simulink model "lcc3_comparison"  (R2024b)
settings: Solver=VariableStepAuto  StartTime=0.0  StopTime=0.016  RelTol=1e-3
InitFcn:
  | SIMSTEP=1e-8; Vin=50; Cs=135e-9; Ls=4.7e-6; Cp=27e-9; fs=280e3; Ron=1.0000000000000001e-05; Rd=1.0000000000000001e-05; Co=6.25e-6; td=0; Coss=0; n=4;
undefined symbols (not defined in the file): Vo_test
libraries: fl_lib x29, nesl_utility x21, ee_lib x15, spsOnDelayLib x6, spsMeanLib x2, spspowerguiLib x1
settings Model: Creator=amazing  LastModifiedBy=amazing

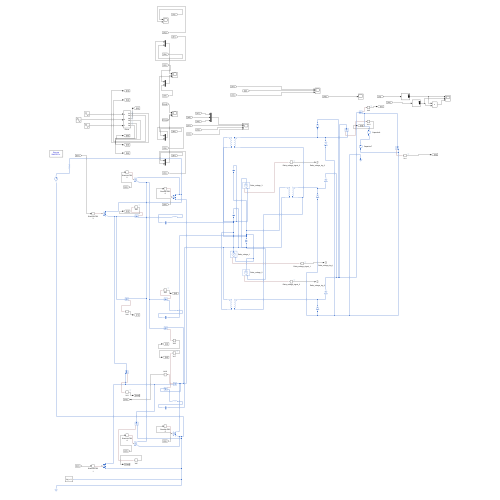
[thumbnail: Simulink's stored preview of the top-level diagram]
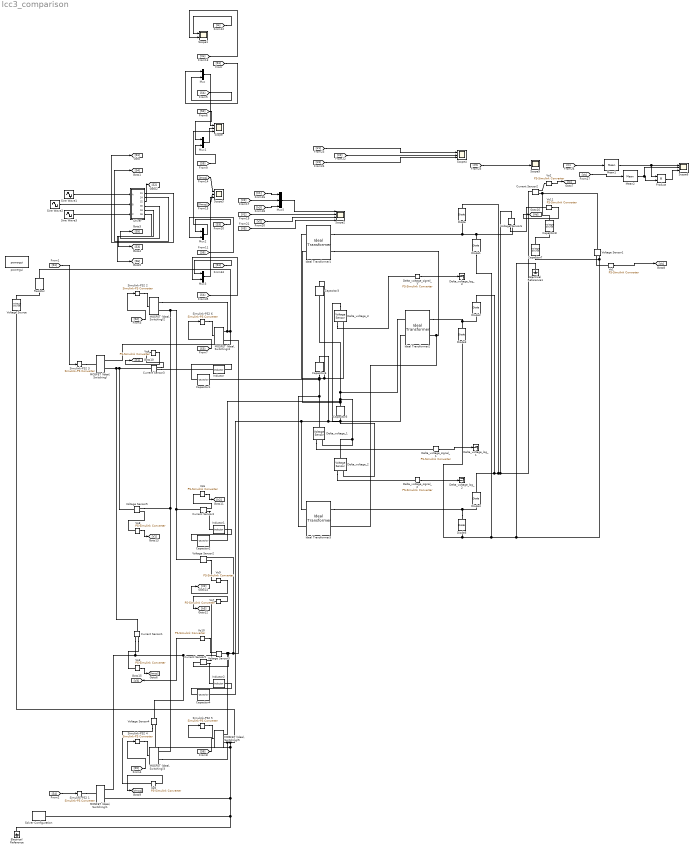
== system lcc3_comparison ==
  Capacitor1 : fl_lib/Electrical/Electrical Elements/Capacitor  c=Cs F  r=1.0000000000000001e-05 Ohm  g=0 1/Ohm  i_specify=off  i_priority=None  i=0 A  i_nominal_specify=off  i_nominal_value=1  i_nominal_unit=A  v_specify=off  v_priority=None  v=0 V  v_nominal_specify=off  v_nominal_value=1  v_nominal_unit=V  vc_specify=on  vc_priority=High  vc=0 V  vc_nominal_specify=off  vc_nominal_value=1  vc_nominal_unit=V
  Capacitor2 : fl_lib/Electrical/Electrical Elements/Capacitor  c=Cs F  r=1.0000000000000001e-05 Ohm  g=0 1/Ohm  i_specify=off  i_priority=None  i=0 A  i_nominal_specify=off  i_nominal_value=1  i_nominal_unit=A  v_specify=off  v_priority=None  v=0 V  v_nominal_specify=off  v_nominal_value=1  v_nominal_unit=V  vc_specify=on  vc_priority=High  vc=0 V  vc_nominal_specify=off  vc_nominal_value=1  vc_nominal_unit=V
  Capacitor3 : fl_lib/Electrical/Electrical Elements/Capacitor  c=Cp F  r=1.0000000000000001e-05 Ohm  g=0 1/Ohm  i_specify=off  i_priority=None  i=0 A  i_nominal_specify=off  i_nominal_value=1  i_nominal_unit=A  v_specify=off  v_priority=None  v=0 V  v_nominal_specify=off  v_nominal_value=1  v_nominal_unit=V  vc_specify=on  vc_priority=High  vc=0 V  vc_nominal_specify=off  vc_nominal_value=1  vc_nominal_unit=V
  Capacitor4 : fl_lib/Electrical/Electrical Elements/Capacitor  c=Cs F  r=1.0000000000000001e-05 Ohm  g=0 1/Ohm  i_specify=off  i_priority=None  i=0 A  i_nominal_specify=off  i_nominal_value=1  i_nominal_unit=A  v_specify=off  v_priority=None  v=0 V  v_nominal_specify=off  v_nominal_value=1  v_nominal_unit=V  vc_specify=on  vc_priority=High  vc=0 V  vc_nominal_specify=off  vc_nominal_value=1  vc_nominal_unit=V
  Capacitor5 : fl_lib/Electrical/Electrical Elements/Capacitor  c=Cp F  r=1.0000000000000001e-05 Ohm  g=0 1/Ohm  i_specify=off  i_priority=None  i=0 A  i_nominal_specify=off  i_nominal_value=1  i_nominal_unit=A  v_specify=off  v_priority=None  v=0 V  v_nominal_specify=off  v_nominal_value=1  v_nominal_unit=V  vc_specify=on  vc_priority=High  vc=0 V  vc_nominal_specify=off  vc_nominal_value=1  vc_nominal_unit=V
  Capacitor6 : fl_lib/Electrical/Electrical Elements/Capacitor  c=Cp F  r=1.0000000000000001e-05 Ohm  g=0 1/Ohm  i_specify=off  i_priority=None  i=0 A  i_nominal_specify=off  i_nominal_value=1  i_nominal_unit=A  v_specify=off  v_priority=None  v=0 V  v_nominal_specify=off  v_nominal_value=1  v_nominal_unit=V  vc_specify=on  vc_priority=High  vc=0 V  vc_nominal_specify=off  vc_nominal_value=1  vc_nominal_unit=V
  Capacitor7 : ee_lib/Sources/Voltage Source  dc_voltage=Vo_test/2 V  ac_voltage=0 V  ac_shift=0 rad  ac_frequency=60 Hz  noise_mode=ee.enum.sources.noise.Disabled  PSD=0 V^2/Hz  sample_time=1e-3 s  repeatability=ee.enum.sources.repeatability.NotRepeatable  user_seed=0  auto_seed=3890346746  i_specify=off  i_priority=None  i=0 A  i_nominal_specify=off  i_nominal_value=1  i_nominal_unit=A  v_specify=off  v_priority=None  v=0 V  v_nominal_specify=off  v_nominal_value=1  v_nominal_unit=V
  Capacitor8 : ee_lib/Sources/Voltage Source  dc_voltage=Vo_test/2 V  ac_voltage=0 V  ac_shift=0 rad  ac_frequency=60 Hz  noise_mode=ee.enum.sources.noise.Disabled  PSD=0 V^2/Hz  sample_time=1e-3 s  repeatability=ee.enum.sources.repeatability.NotRepeatable  user_seed=0  auto_seed=3499211588  i_specify=off  i_priority=None  i=0 A  i_nominal_specify=off  i_nominal_value=1  i_nominal_unit=A  v_specify=off  v_priority=None  v=0 V  v_nominal_specify=off  v_nominal_value=1  v_nominal_unit=V
  Current Sensor{1..5} (5 alike) : fl_lib/Electrical/Electrical Sensors/Current Sensor
  Delta_voltage_1 : fl_lib/Electrical/Electrical Sensors/Voltage Sensor
  Delta_voltage_2 : fl_lib/Electrical/Electrical Sensors/Voltage Sensor
  Delta_voltage_3 : fl_lib/Electrical/Electrical Sensors/Voltage Sensor
  Delta_voltage_log_1 : Terminator
  Delta_voltage_log_2 : Terminator
  Delta_voltage_log_3 : Terminator
  Delta_voltage_signal_1 : nesl_utility/PS-Simulink Converter  PhysicalDomain=network_engine_domain  SubClassName=ps_output  LeftPortType=input  RightPortType=output  PseudoPeriodic=off  Frequencies=[]  VectorFormat=inherit  Unit=inherit  AffineConversion=off
  Delta_voltage_signal_2 : nesl_utility/PS-Simulink Converter  PhysicalDomain=network_engine_domain  SubClassName=ps_output  LeftPortType=input  RightPortType=output  PseudoPeriodic=off  Frequencies=[]  VectorFormat=inherit  Unit=inherit  AffineConversion=off
  Delta_voltage_signal_3 : nesl_utility/PS-Simulink Converter  PhysicalDomain=network_engine_domain  SubClassName=ps_output  LeftPortType=input  RightPortType=output  PseudoPeriodic=off  Frequencies=[]  VectorFormat=inherit  Unit=inherit  AffineConversion=off
  Diode{,1..5} (6 alike) : ee_lib/Semiconductors & Converters/Diode  ModelType=ee.enum.diode.modelType.pwl  TableType=ee.enum.diode.tableType.IfMat  IfMat=[.07, .12, .19, 1.75, 4.24, 7.32, 11.2; .16, .3, .72, 2.14, 5.02, 8.35, 13.12] A  VfMat=[.9, 1.15, 1.25, 1.5, 1.75, 2.17, 2.6, 2.85; .58, .68, .75, 1.1, 1.38, 1.77, 2.27, 2.7] V  TjVec=[25, 125] degC  VfVec=[.5, .7, .9, 1.3, 1.7, 2.1, 2.5] V  IfVec=[.1, .2, .5, 1, 2, 4, 7, 10] A  IrMat=[1e-06, 2e-06, 5e-06, 1e-05, 2.5e-05, 5e-05, .0001; 2e-06, 5e-06, 1e-05, 4e-05, 8e-05, .0002, .0005] A  VrMat=[10, 100, 200, 250, 300, 325, 350; 10, 70, 160, 220, 270, 300, 320] V  VrVec=[10, 20, 40, 50, 70, 80, 100] V  IrVec=[1e-06, 2e-06, 5e-06, 1e-05, 2e-05, 5e-05, .0001] A  Vf=9.9999999999999995e-07 V  Ron=1.0000000000000001e-05 Ohm  Goff=1e-10 S  prmExp=ee.enum.diode.expParam.useTwo  I12=[.0137, .545] A  V12=[.6, .7] V  RS=0 Ohm  Tmeas=298.15 K  IS=1e-12 A  ec=1  I1=0.0137 A  V1=0.6 V  N_series=1  N_parallel=1  ZenerEnable=false  Rz=0.3 Ohm  BV=inf V  C_param=ee.enum.diode.capParam.fixed  CJ=0 pF  CJ0=5 pF  Vvec=[.1, 10, 100] V  Cvec=[3.5, 1, .4] pF  VJ=1 V  Mgrad=0.5  FC=0.5  Q_param=ee.enum.diode.recoveryParam.off  iRM=-7.15 A  iF=4 A  didt=-750 A/us  trr_factor=3  trr=115 ns  Qrr=150 nA*s  Vr=-600 V  Ls=150 nH  Erec=0.03 J  TT=50 ns  tau=100 ns  T_param=ee.enum.diode.temperatureParam.off  Tdevice=298.15 K  I1_T2=0.245 A  V1_T2=0.5 V  IS_T2=1.25e-7 A  Tmeas2=125 degC  XTI_param=ee.enum.diode.xtiParam.pn  XTI=3  EG_param=ee.enum.diode.egapParam.material_si  EG=1.11 eV  dBVdT=0 V/K  fault_action=simscape.enum.assert.action.none  t_fault=inf s  enable_fault_input=simscape.enum.onoff.off  i_specify=off  i_priority=None  i=0 A  i_nominal_specify=off  i_nominal_value=1  i_nominal_unit=A  v_specify=off  v_priority=None  v=0 V  v_nominal_specify=off  v_nominal_value=1  v_nominal_unit=V  v_capacitor_specify=off  v_capacitor_priority=None  v_capacitor=0 V  v_capacitor_nominal_specify=off  v_capacitor_nominal_value=1  v_capacitor_nominal_unit=V  Qj_specify=off  Qj_priority=High  Qj=0 C  Qj_nominal_specify=off  Qj_nominal_value=1  Qj_nominal_unit=C  i_diode_specify=off  i_diode_priority=None  i_diode=0 A  i_diode_nominal_specify=off  i_diode_nominal_value=1  i_diode_nominal_unit=A  v_diode_specify=off  v_diode_priority=None  v_diode=0 V  v_diode_nominal_specify=off  v_diode_nominal_value=1  v_diode_nominal_unit=V  i_capacitor_specify=off  i_capacitor_priority=None  i_capacitor=0 A  i_capacitor_nominal_specify=off  i_capacitor_nominal_value=1  i_capacitor_nominal_unit=A  power_dissipated_specify=off  power_dissipated_priority=None  power_dissipated=0 W  power_dissipated_nominal_specify=off  power_dissipated_nominal_value=1  power_dissipated_nominal_unit=W  fidelity_level=ee.enum.diode.fidelity.includeChargeDyn  rec_loss_model=ee.enum.diode.reverseRecoveryModel.fixed  ErecVal=0 J  scaleWithIandV=true  ErecMat=zeros(2, 3) J  TjrecVec=[298.15, 398.15] K  IfrecVec=[.1, 1, 10] A  IrecVal=10 A  VrecVal=10 V  tFilter=1 / 1000 / 100 s  thermal_network_parameterization=ee.enum.thermalNetworkTopology.junctionCase  Rth=[0, 10] K/W  Rth_Cauer=[1, 3, 10] K/W  Rth_Foster=[.08, .14, .22, .16] K/W  thermal_mass_parameterization=ee.enum.thermalNetwork.timeconstant  thermal_mass=[0, 1] J/K  thermal_mass_Cauer=[.1, .3, 1] J/K  thermal_mass_Foster=[.001, .005, .05, .5] J/K  thermal_time_constant=[0, 10] s  thermal_time_constant_Cauer=[1, 3, 10] s  thermal_time_constant_Foster=[7e-05, .0007, .01, .08] s  thermal_mass_initial_temperatures=[25, 25] degC  thermal_mass_initial_temperatures_Cauer=[25, 25, 25] degC  junction_thermal_mass=0.01 J/K  Tvec_initial_Foster=[25, 25, 25, 25] degC  no_thermal_network=0  junction_temperature_specify=off  junction_temperature_priority=None  junction_temperature=25 degC  junction_temperature_nominal_specify=off  junction_temperature_nominal_value=1  junction_temperature_nominal_unit=degC
  Driver : Subsystem
  Electrical Reference : fl_lib/Electrical/Electrical Elements/Electrical Reference
  Electrical Reference1 : fl_lib/Electrical/Electrical Elements/Electrical Reference
  Ideal Transformer1 : fl_lib/Electrical/Electrical Elements/Ideal Transformer  n=1/n  i1_specify=off  i1_priority=None  i1=0 A  i1_nominal_specify=off  i1_nominal_value=1  i1_nominal_unit=A  v1_specify=off  v1_priority=None  v1=0 V  v1_nominal_specify=off  v1_nominal_value=1  v1_nominal_unit=V  i2_specify=off  i2_priority=None  i2=0 A  i2_nominal_specify=off  i2_nominal_value=1  i2_nominal_unit=A  v2_specify=off  v2_priority=None  v2=0 V  v2_nominal_specify=off  v2_nominal_value=1  v2_nominal_unit=V
  Ideal Transformer2 : fl_lib/Electrical/Electrical Elements/Ideal Transformer  n=1/n  i1_specify=off  i1_priority=None  i1=0 A  i1_nominal_specify=off  i1_nominal_value=1  i1_nominal_unit=A  v1_specify=off  v1_priority=None  v1=0 V  v1_nominal_specify=off  v1_nominal_value=1  v1_nominal_unit=V  i2_specify=off  i2_priority=None  i2=0 A  i2_nominal_specify=off  i2_nominal_value=1  i2_nominal_unit=A  v2_specify=off  v2_priority=None  v2=0 V  v2_nominal_specify=off  v2_nominal_value=1  v2_nominal_unit=V
  Ideal Transformer3 : fl_lib/Electrical/Electrical Elements/Ideal Transformer  n=1/n  i1_specify=off  i1_priority=None  i1=0 A  i1_nominal_specify=off  i1_nominal_value=1  i1_nominal_unit=A  v1_specify=off  v1_priority=None  v1=0 V  v1_nominal_specify=off  v1_nominal_value=1  v1_nominal_unit=V  i2_specify=off  i2_priority=None  i2=0 A  i2_nominal_specify=off  i2_nominal_value=1  i2_nominal_unit=A  v2_specify=off  v2_priority=None  v2=0 V  v2_nominal_specify=off  v2_nominal_value=1  v2_nominal_unit=V
  Inductor : fl_lib/Electrical/Electrical Elements/Inductor  l=Ls H  r=1.0000000000000001e-05 Ohm  g=1e-10 1/Ohm  i_specify=off  i_priority=None  i=0 A  i_nominal_specify=off  i_nominal_value=1  i_nominal_unit=A  v_specify=off  v_priority=None  v=0 V  v_nominal_specify=off  v_nominal_value=1  v_nominal_unit=V  i_L_specify=on  i_L_priority=High  i_L=0 A  i_L_nominal_specify=off  i_L_nominal_value=1  i_L_nominal_unit=A
  Inductor1 : fl_lib/Electrical/Electrical Elements/Inductor  l=Ls H  r=1.0000000000000001e-05 Ohm  g=1e-10 1/Ohm  i_specify=off  i_priority=None  i=0 A  i_nominal_specify=off  i_nominal_value=1  i_nominal_unit=A  v_specify=off  v_priority=None  v=0 V  v_nominal_specify=off  v_nominal_value=1  v_nominal_unit=V  i_L_specify=on  i_L_priority=High  i_L=0 A  i_L_nominal_specify=off  i_L_nominal_value=1  i_L_nominal_unit=A
  Inductor2 : fl_lib/Electrical/Electrical Elements/Inductor  l=Ls H  r=1.0000000000000001e-05 Ohm  g=1e-10 1/Ohm  i_specify=off  i_priority=None  i=0 A  i_nominal_specify=off  i_nominal_value=1  i_nominal_unit=A  v_specify=off  v_priority=None  v=0 V  v_nominal_specify=off  v_nominal_value=1  v_nominal_unit=V  i_L_specify=on  i_L_priority=High  i_L=0 A  i_L_nominal_specify=off  i_L_nominal_value=1  i_L_nominal_unit=A
  MOSFET (Ideal, Switching){,1..5} (6 alike) : ee_lib/Semiconductors & Converters/MOSFET (Ideal, Switching)  port_option=ee.enum.controlport.ps  Rds=1.0000000000000001e-05 Ohm  Goff=1e-10 1/Ohm  Vth=2 V  diode_param=ee.enum.semiconductors.protectionDiode.external  diode_Vf=1e-9 V  diode_Ron=1e-9 Ohm  diode_Goff=1e-12 1/Ohm  diode_C=50e-9 F  diode_iRM=-235 A  diode_iF=300 A  diode_idot=-50 A/us  diode_trr_param=ee.enum.converters.diodeReverseParam.trr_factor  diode_trr_factor=3  diode_trr=15 us  diode_Qrr=1500 s*uA  ids_specify=off  ids_priority=None  ids=0 A  ids_nominal_specify=off  ids_nominal_value=1  ids_nominal_unit=A  vds_specify=off  vds_priority=None  vds=0 V  vds_nominal_specify=off  vds_nominal_value=1  vds_nominal_unit=V  vgs_specify=off  vgs_priority=None  vgs=0 V  vgs_nominal_specify=off  vgs_nominal_value=1  vgs_nominal_unit=V  thermal_loss_option=ee.enum.converters.thermalLossOption.constantvalues  Von_data=[0, 1.8, 3.2, 6, 10, 16; 0, 2, 5.5, 9.5, 15, 25] V  Tj=[298.15, 448.15] K  Iout_data=[0, 20, 40, 60, 80, 100] A  Eon_data=[0, 55.04, 124.57, 235.53, 362.12; 0, 71.25, 161.25, 304.88, 468.75] * 1e-6 J  Eoff_data=[0, 18, 30, 56.1, 76.5; 0, 22.5, 37.5, 70.13, 95.63] * 1e-6 J  Eon_data_3D=[zeros(2, 5, 3)] J  Eoff_data_3D=[zeros(2, 5, 3)] J  Tj_loss=[298.15, 448.15] K  Iout_data_loss=[0, 10, 20, 30, 40] A  tabulateWithVds=false  Vds_loss=[0, 150, 300] V  Eon_scalar=22.86e-3 J  Eoff_scalar=17.14e-3 J  Voff=300 V  Iout_scalar=600 A  useCurrentFromPreviousCycle=false  useVoltageFromPreviousCycle=false  diodeModelType=ee.enum.converters.diodeModelType.pwl  diodeTableType=ee.enum.diode.tableType.IfMat  diode_ReverseIVType=ee.enum.diode.diodeReverseIV.constant  diode_IfMat=[.07, .12, .19, 1.75, 4.24, 7.32, 11.2; .16, .3, .72, 2.14, 4.02, 6.35, 9.12] A  diode_VfMat=[.9, 1.15, 1.25, 1.5, 1.75, 2.17, 2.6, 2.85; .58, .68, .75, 1.1, 1.38, 1.77, 2.27, 2.7] V  diode_TjVec=[25, 125] degC  diode_VfVec=[.5, .7, .9, 1.3, 1.7, 2.1, 2.5] V  diode_IfVec=[.1, .2, .5, 1, 2, 4, 7, 10] A  diode_IrMat=[1e-06, 2e-06, 5e-06, 1e-05, 2.5e-05, 5e-05, .0001; 2e-06, 5e-06, 1e-05, 4e-05, 8e-05, .0002, .0005] A  diode_VrMat=[10, 100, 200, 250, 300, 325, 350; 10, 70, 160, 220, 270, 300, 320] V  diode_VrVec=[10, 20, 40, 50, 70, 80, 100] V  diode_IrVec=[1e-06, 2e-06, 5e-06, 1e-05, 2e-05, 5e-05, .0001] A  diode_Vr=-600 V  diode_Ls=150 nH  diode_Erec=0.03 J  diode_rec_loss_model=ee.enum.diode.reverseRecoveryModel.fixed  diode_ErecVal=0 J  diode_scaleWithIandV=true  diode_ErecMat=zeros(2, 3) J  diode_TjrecVec=[298.15, 398.15] K  diode_IfrecVec=[.1, 1, 10] A  diode_IrecVal=10 A  diode_VrecVal=10 V  diode_tFilter=1 / 1000 / 100 s  separateThermalPortForDiode=false  thermal_network_parameterization=ee.enum.thermalNetworkTopology.external  Rth=[.03, .2] K/W  Rth_Cauer=[.03, .1, .2] K/W  Rth_Foster=[.08, .14, .22, .16] K/W  thermal_mass_parameterization=ee.enum.thermalNetwork.timeconstant  thermal_mass=[3, 25] J/K  thermal_mass_Cauer=[3, 10, 25] J/K  thermal_mass_Foster=[.001, .005, .05, .5] J/K  thermal_time_constant=[.1, 5] s  thermal_time_constant_Cauer=[.1, 1, 5] s  thermal_time_constant_Foster=[7e-05, .0007, .01, .08] s  thermal_mass_initial_temperatures=[25, 25] degC  thermal_mass_initial_temperatures_Cauer=[25, 25, 25] degC  junction_thermal_mass=0.1 J/K  Tvec_initial_Foster=[25, 25, 25, 25] degC  RthDiode=[.03, .2] K/W  RthCauerDiode=[.03, .1, .2] K/W  RthFosterDiode=[.03, .2] K/W  thermalMassDiode=[3, 25] J/K  thermalMassCauerDiode=[3, 10, 25] J/K  thermalMassFosterDiode=[33, 50] J/K  thermalTauDiode=[.1, 5] s  thermalTauCauerDiode=[.1, 1, 5] s  thermalTauFosterDiode=[1, 10] s  thermalMassInitTempDiode=[25, 25] degC  thermalMassInitTempCauerDiode=[25, 25, 25] degC  junctionthermalMassDiode=0.1 J/K  TVecInitialFosterDiode=[25, 25, 25, 25] degC  no_thermal_network=0  mosfet_junction_temperature_specify=off  mosfet_junction_temperature_priority=None  mosfet_junction_temperature=25 degC  mosfet_junction_temperature_nominal_specify=off  mosfet_junction_temperature_nominal_value=1  mosfet_junction_temperature_nominal_unit=degC  diode_junction_temperature_specify=off  diode_junction_temperature_priority=None  diode_junction_temperature=25 degC  diode_junction_temperature_nominal_specify=off  diode_junction_temperature_nominal_value=1  diode_junction_temperature_nominal_unit=degC  Qj_specify=off  Qj_priority=None  Qj=0 W  Qj_nominal_specify=off  Qj_nominal_value=1  Qj_nominal_unit=W  accumulatedSwitchingLosses_specify=off  accumulatedSwitchingLosses_priority=None  accumulatedSwitchingLosses=0 J
  Mean1 : spsMeanLib/Mean  Freq=100e3  Vinit=0  Ts=0
  Mean2 : spsMeanLib/Mean  Freq=100e3  Vinit=0  Ts=0
  Mux{,1..3} (4 alike) : Mux  Inputs=2
  Mux5 : Mux  Inputs=3
  Product : Product
  Resistor : fl_lib/Electrical/Electrical Elements/Resistor  R=1.0000000000000001e-05 Ohm  i_specify=off  i_priority=None  i=0 A  i_nominal_specify=off  i_nominal_value=1  i_nominal_unit=A  v_specify=off  v_priority=None  v=0 V  v_nominal_specify=off  v_nominal_value=1  v_nominal_unit=V
  Scope{,3..4,6} (4 alike) : Scope  NumInputPorts=3
  Scope1 : Scope  NumInputPorts=2
  Scope2 : Scope  NumInputPorts=4
  Scope5 : Scope
  Simulink-PS2 {1..6} (6 alike) : nesl_utility/Simulink-PS Converter  PhysicalDomain=network_engine_domain  SubClassName=ps_input  LeftPortType=input  RightPortType=output  PseudoPeriodic=off  Frequencies=[]  NoiseDistribution=none  NoiseParameters=[]  Unit=1  AffineConversion=off  FilteringAndDerivatives=provide  SimscapeFilterOrder=1  InputFilterTimeConstant=0.001  UdotUserProvided=0
  Sine Wave1 : Sin  Frequency=2*pi*fs  SampleTime=0
  Sine Wave2 : Sin  Frequency=2*pi*fs  Phase=2*pi/3  SampleTime=0
  Sine Wave3 : Sin  Frequency=2*pi*fs  Phase=4*pi/3  SampleTime=0
  Solver Configuration : nesl_utility/Solver Configuration  PhysicalDomain=network_engine_domain  SubClassName=solver  LeftPortType=input  RightPortType=generic  Tones=[]  Harmonics=[]  SimulateNoise=off  Profile=off  UseLocalSampling=off  EnableSwitchedLinearOptims=on  FrequencyDomain=off  UseCCode=off  RelTol=0.001  AbsTol=0.001  MinStep=1e-09  ToWorkspace=off  RevertToSquareIcSolve=off  NumHomotopyIterations=100  PhasorMode=off  PhasorModeNumHarmonics=1  ConsistencySolver=NEWTON_XTOL_AFTER_FTOL  IndexReductionMethod=DerivativeReplacement  DoDC=off  ResidualTolerance=1e-09  ConsistencyTolSource=GLOBAL  ConsistencyAbsTol=0.001  ConsistencyRelTol=0.001  ConsistencyTolFactor=0.001  UseLocalSolver=off  LocalSolverChoice=NE_BACKWARD_EULER_ADVANCER  ResolveIndetEquations=on  FunctionEvalNumThread=1  LocalSolverSampleTime=0.001  DoFixedCost=off  MaxNonlinIter=3  MaxModeIter=2  ComputeImpulses=off  ImpulseIterations=2  LinearAlgebra=auto  LinearAlgebraNumThread=0  EquationFormulation=NE_TIME_EF  DelaysMemoryBudget=1024  AutomaticFiltering=on  FilteringTimeConstant=0.001  PartitionStorageMethod=AS_NEEDED  PartitionMemoryBudget=1024  PartitionMethod=ROBUST  MultibodyUseLocalSolver=off  MultibodyLocalSolverChoice=ODE1  MultibodyLocalSolverSampleTime=0.001
  Vo{1..11} (11 alike) : nesl_utility/PS-Simulink Converter  PhysicalDomain=network_engine_domain  SubClassName=ps_output  LeftPortType=input  RightPortType=output  PseudoPeriodic=off  Frequencies=[]  VectorFormat=inherit  Unit=inherit  AffineConversion=off
  Voltage Sensor{1..6} (6 alike) : fl_lib/Electrical/Electrical Sensors/Voltage Sensor
  Voltage Source : ee_lib/Sources/Voltage Source  dc_voltage=Vin V  ac_voltage=0 V  ac_shift=0 rad  ac_frequency=0 Hz  noise_mode=ee.enum.sources.noise.Disabled  PSD=0 V^2/Hz  sample_time=1e-3 s  repeatability=ee.enum.sources.repeatability.NotRepeatable  user_seed=0  auto_seed=3890346746  i_specify=off  i_priority=None  i=0 A  i_nominal_specify=off  i_nominal_value=1  i_nominal_unit=A  v_specify=off  v_priority=None  v=0 V  v_nominal_specify=off  v_nominal_value=1  v_nominal_unit=V
  powergui : spspowerguiLib/powergui  Priority=1  SimulationMode=Discrete  SampleTime=SIMSTEP  frequency=60  Iterations=50  frequencyindice=60  Pbase=100e6  ErrMax=1e-4  UnitsV=kV  UnitsW=MW  buscounter=0  FunctionMessages=off  echomessages=off  EnableUseOfTLC=off  CurrentSourceSwitches=off  DisableSnubberDevices=off  DisableRonSwitches=off  DisableVfSwitches=off  DisplayEquations=off  AutomaticDiscreteSolvers=off  SolverType=Tustin/Backward Euler (TBE)  Interpol=off  ExternalGateDelay=off  methode=off  Ts=100  x0status=blocks  SPID=on  SwTol=0  HookPort=off  NonlinearTolerance=1e-4  nMaxIteration=100  ContinueOnMaxIteration=off  RestoreLinks=warning  ResistiveCurrentMeasurement=off  Frange=[0:2:500]  Ylog=off  Xlog=on  ShowGrid=off  save=off  variable=ZData  structure=0  ZoomFFT=off  StartTime=0.0  cycles=1  DisplayStyle=1  fundamental=60  FreqAxis=off  MaxFrequency=1000  frequencyindicesteady=1  RmsSteady=1  display=off
  wires:
  Delta_voltage_signal_3/1 -> Delta_voltage_log_3/1
  Delta_voltage_signal_2/1 -> Delta_voltage_log_2/1
  Delta_voltage_signal_1/1 -> Delta_voltage_log_1/1
  [S1] -> Mux3/1
  [S4] -> Mux3/2
  Mux3/1 -> Scope3/3
  [Vd] -> Scope5/1
  Vo11/1 -> [Vd]
  Product/1 -> Scope6/3
  Mean2/1 -> Scope6/2, Product/2
  [Vo] -> Mean2/1
  Mean1/1 -> Product/1, Scope6/1
  [Io] -> Mean1/1
  [Ir3] -> Scope4/3
  [Ir1] -> Scope4/1
  [Ir2] -> Scope4/2
  [Vmos] -> Scope3/2
  [Imos] -> Scope3/1
  Vo5/1 -> [Vmos]
  [S5] -> Simulink-PS2 4/1
  Vo3/1 -> [Imos]
  [Vo] -> Scope1/2
  [Io] -> Scope1/1
  Mux5/1 -> Scope2/1
  [V2] -> Scope2/3
  [V3] -> Scope2/4
  [V1] -> Scope2/2
  Vo10/1 -> [V3]
  Vo9/1 -> [V2]
  Vo8/1 -> [V1]
  [Ir3] -> Mux5/3
  [Ir2] -> Mux5/2
  [Ir1] -> Mux5/1
  Vo7/1 -> [Ir3]
  Vo6/1 -> [Ir2]
  Vo4/1 -> [Ir1]
  Mux2/1 -> Scope/3
  Mux/1 -> Scope/1
  Mux1/1 -> Scope/2
  [S6] -> Mux2/2
  [S3] -> Mux2/1
  [S2] -> Mux1/1
  [S5] -> Mux1/2
  [S4] -> Mux/2
  [S1] -> Mux/1
  Vo2/1 -> [Io]
  Vo1/1 -> [Vo]
  [S3] -> Simulink-PS2 6/1
  [S6] -> Simulink-PS2 5/1
  [S2] -> Simulink-PS2 2/1
  [S4] -> Simulink-PS2 1/1
  [S1] -> Simulink-PS2 3/1
  Driver/6(S6) -> [S6]
  Driver/5(S3) -> [S3]
  Driver/4(S5) -> [S5]
  Driver/3(S2) -> [S2]
  Sine Wave3/1 -> Driver/3(C)
  Sine Wave2/1 -> Driver/2(B)
  Driver/2(S4) -> [S4]
  Sine Wave1/1 -> Driver/1(A)
  Driver/1(S1) -> [S1]
  connections:
  Delta_voltage_3/RConn1 -- Delta_voltage_signal_3/LConn1
  Delta_voltage_2/RConn1 -- Delta_voltage_signal_2/LConn1
  Delta_voltage_1/RConn1 -- Delta_voltage_signal_1/LConn1
  Capacitor7/LConn1 -- Capacitor8/RConn1
  Current Sensor2/RConn2 -- Voltage Sensor1/LConn1 -- Capacitor8/LConn1
  Voltage Sensor6/RConn1 -- Vo11/LConn1
  Vo6/LConn1 -- Current Sensor4/RConn1
  Voltage Sensor4/RConn1 -- Vo5/LConn1
  Current Sensor1/RConn1 -- Vo3/LConn1
  "MOSFET (Ideal, Switching)1"/RConn1 -- Voltage Sensor3/RConn2 -- Voltage Sensor4/LConn1 -- Current Sensor1/RConn2
  Vo10/LConn1 -- Voltage Sensor3/RConn1
  Voltage Sensor2/RConn1 -- Vo9/LConn1
  Vo8/LConn1 -- Voltage Sensor5/RConn1
  Current Sensor5/RConn1 -- Vo7/LConn1
  Current Sensor5/RConn2 -- Inductor2/LConn1
  Current Sensor4/RConn2 -- Inductor1/LConn1
  Current Sensor3/RConn1 -- Vo4/LConn1
  Current Sensor3/RConn2 -- Inductor/LConn1
  Ideal Transformer1/RConn2 -- Ideal Transformer2/RConn2 -- Ideal Transformer3/RConn2
  Current Sensor2/RConn1 -- Vo2/LConn1
  Diode2/RConn1 -- Current Sensor2/LConn1 -- Voltage Sensor6/LConn1 -- Diode/RConn1 -- Diode4/RConn1
  Vo1/LConn1 -- Voltage Sensor1/RConn1
  Diode3/LConn1 -- Electrical Reference1/LConn1 -- Voltage Sensor1/RConn2 -- Capacitor7/RConn1 -- Diode1/LConn1 -- Diode5/LConn1
  Delta_voltage_3/LConn1 -- Ideal Transformer3/LConn1 -- Capacitor4/RConn1 -- Capacitor6/LConn1 -- Capacitor5/RConn1 -- Ideal Transformer2/LConn2 -- Delta_voltage_2/RConn2
  Capacitor2/LConn1 -- Inductor1/RConn1
  Capacitor1/LConn1 -- Inductor/RConn1
  Current Sensor5/LConn1 -- Voltage Sensor2/RConn2 -- "MOSFET (Ideal, Switching)4"/RConn2 -- Voltage Sensor3/LConn1 -- "MOSFET (Ideal, Switching)5"/RConn1
  Capacitor5/LConn1 -- Delta_voltage_1/RConn2 -- Delta_voltage_2/LConn1 -- Ideal Transformer2/LConn1 -- Capacitor3/RConn1 -- Capacitor2/RConn1 -- Ideal Transformer1/LConn2
  Delta_voltage_3/RConn2 -- Capacitor6/RConn1 -- Ideal Transformer3/LConn2 -- Delta_voltage_1/LConn1 -- Capacitor1/RConn1 -- Ideal Transformer1/LConn1 -- Capacitor3/LConn1
  Diode5/RConn1 -- Ideal Transformer3/RConn1 -- Diode4/LConn1
  Ideal Transformer2/RConn1 -- Diode3/RConn1 -- Diode2/LConn1
  Voltage Sensor6/RConn2 -- Ideal Transformer1/RConn1 -- Diode/LConn1 -- Diode1/RConn1
  "MOSFET (Ideal, Switching)4"/RConn1 -- Resistor/RConn1 -- "MOSFET (Ideal, Switching)"/RConn1 -- "MOSFET (Ideal, Switching)2"/RConn1
  "MOSFET (Ideal, Switching)5"/RConn2 -- Electrical Reference/LConn1 -- Solver Configuration/RConn1 -- "MOSFET (Ideal, Switching)1"/RConn2 -- Voltage Sensor4/RConn2 -- Voltage Source/RConn1 -- "MOSFET (Ideal, Switching)3"/RConn2
  Resistor/LConn1 -- Voltage Source/LConn1
  Capacitor4/LConn1 -- Inductor2/RConn1
  Voltage Sensor5/RConn2 -- Current Sensor4/LConn1 -- Voltage Sensor2/LConn1 -- "MOSFET (Ideal, Switching)2"/RConn2 -- "MOSFET (Ideal, Switching)3"/RConn1
  Current Sensor3/LConn1 -- "MOSFET (Ideal, Switching)"/RConn2 -- Current Sensor1/LConn1 -- Voltage Sensor5/LConn1
  Simulink-PS2 6/RConn1 -- "MOSFET (Ideal, Switching)4"/LConn1
  Simulink-PS2 5/RConn1 -- "MOSFET (Ideal, Switching)5"/LConn1
  Simulink-PS2 4/RConn1 -- "MOSFET (Ideal, Switching)3"/LConn1
  Simulink-PS2 2/RConn1 -- "MOSFET (Ideal, Switching)2"/LConn1
  Simulink-PS2 1/RConn1 -- "MOSFET (Ideal, Switching)1"/LConn1
  Simulink-PS2 3/RConn1 -- "MOSFET (Ideal, Switching)"/LConn1

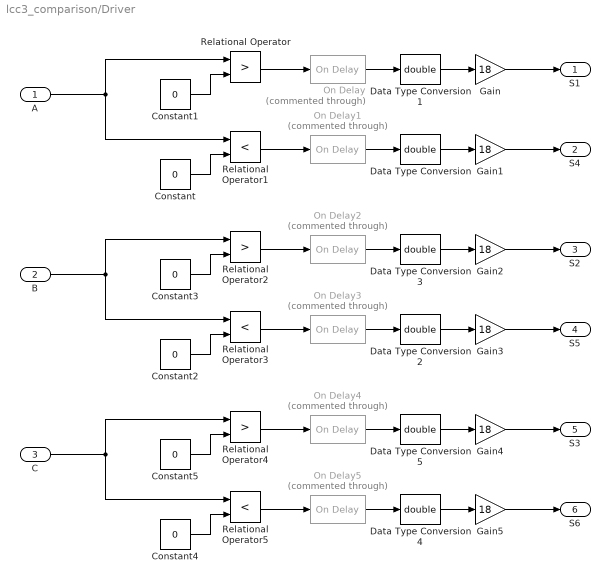
== system lcc3_comparison/Driver ==
  A : Inport
  B : Inport  Port=2
  C : Inport  Port=3
  Constant{,1..5} (6 alike) : Constant  Value=0
  Data Type Conversion{,1..5} (6 alike) : DataTypeConversion  OutDataTypeStr=double  SaturateOnIntegerOverflow=off  RndMeth=Floor
  Gain{,1..5} (6 alike) : Gain  Gain=18
  On Delay{,1..5} (6 alike) : spsOnDelayLib/On Delay  Commented=through  DelayType=On delay  delay=td  ic=0  Ts=0
  Relational Operator : RelationalOperator  Operator=>  OutDataTypeStr=boolean  RndMeth=Simplest  InputSameDT=off
  Relational Operator1 : RelationalOperator  Operator=<  OutDataTypeStr=boolean  RndMeth=Simplest  InputSameDT=off
  Relational Operator2 : RelationalOperator  Operator=>  OutDataTypeStr=boolean  RndMeth=Simplest  InputSameDT=off
  Relational Operator3 : RelationalOperator  Operator=<  OutDataTypeStr=boolean  RndMeth=Simplest  InputSameDT=off
  Relational Operator4 : RelationalOperator  Operator=>  OutDataTypeStr=boolean  RndMeth=Simplest  InputSameDT=off
  Relational Operator5 : RelationalOperator  Operator=<  OutDataTypeStr=boolean  RndMeth=Simplest  InputSameDT=off
  S1 : Outport
  S4 : Outport  Port=2
  S2 : Outport  Port=3
  S5 : Outport  Port=4
  S3 : Outport  Port=5
  S6 : Outport  Port=6
  wires:
  On Delay/1 -> Data Type Conversion1/1
  Relational Operator1/1 -> On Delay1/1
  Constant1/1 -> Relational Operator/2
  On Delay1/1 -> Data Type Conversion/1
  Relational Operator/1 -> On Delay/1
  Constant/1 -> Relational Operator1/2
  A/1 -> Relational Operator1/1, Relational Operator/1
  Data Type Conversion/1 -> Gain1/1
  Data Type Conversion1/1 -> Gain/1
  Gain/1 -> S1/1
  Gain1/1 -> S4/1
  Data Type Conversion2/1 -> Gain3/1
  Relational Operator2/1 -> On Delay2/1
  B/1 -> Relational Operator3/1, Relational Operator2/1
  Data Type Conversion3/1 -> Gain2/1
  On Delay2/1 -> Data Type Conversion3/1
  Gain3/1 -> S5/1
  Relational Operator3/1 -> On Delay3/1
  Gain2/1 -> S2/1
  On Delay3/1 -> Data Type Conversion2/1
  Constant2/1 -> Relational Operator3/2
  Constant3/1 -> Relational Operator2/2
  Data Type Conversion4/1 -> Gain5/1
  Relational Operator4/1 -> On Delay4/1
  C/1 -> Relational Operator5/1, Relational Operator4/1
  Data Type Conversion5/1 -> Gain4/1
  On Delay4/1 -> Data Type Conversion5/1
  Gain5/1 -> S6/1
  Relational Operator5/1 -> On Delay5/1
  Gain4/1 -> S3/1
  On Delay5/1 -> Data Type Conversion4/1
  Constant4/1 -> Relational Operator5/2
  Constant5/1 -> Relational Operator4/2
